simulink model "WBR_Simulator"  (R2023b)
settings: Solver=FixedStepAuto  StartTime=0.0  StopTime=60  FixedStep=0.001  MaxStep=0.001
undefined symbols (not defined in the file or in its folder): DiscIntNeverNeededParam, magnitude, robot_stats, SIMPARAM, X, Y, Z
libraries: sm_lib x73, nesl_utility x50, simulink x17, slpidlib x6, dsparch4 x2
(part 1 of 7)
settings Model: Creator=User  LastModifiedBy=User

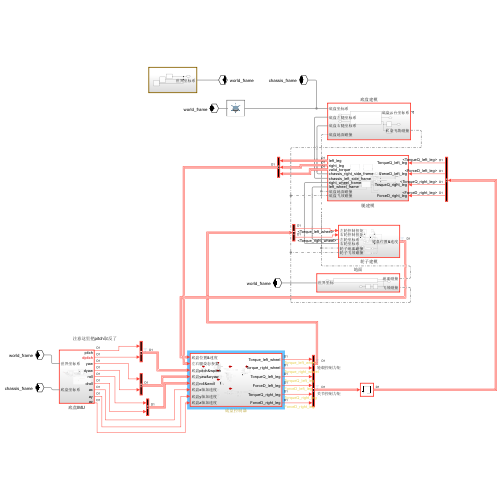
[thumbnail: Simulink's stored preview of the top-level diagram]
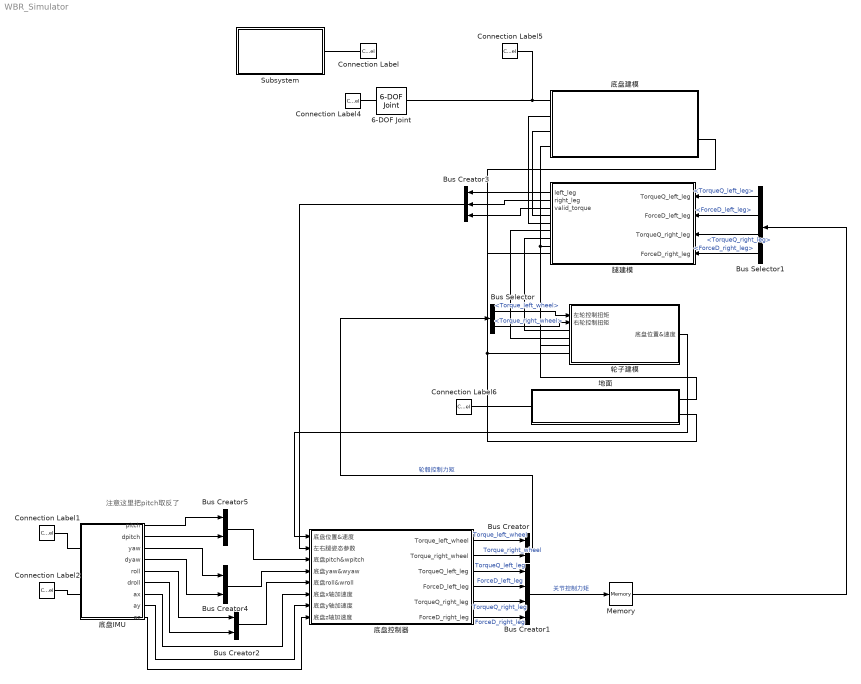
== system WBR_Simulator ==
  note: 注意这里把pitch取反了
  6-DOF Joint : sm_lib/Joints/6-DOF Joint  JointMode=Normal  SenseConstraintForce=off  SenseConstraintForceX=off  SenseConstraintForceY=off  SenseConstraintForceZ=off  SenseConstraintTorque=off  SenseConstraintTorqueX=off  SenseConstraintTorqueY=off  SenseConstraintTorqueZ=off  SenseTotalForce=off  SenseTotalForceX=off  SenseTotalForceY=off  SenseTotalForceZ=off  SenseTotalTorque=off  SenseTotalTorqueX=off  SenseTotalTorqueY=off  SenseTotalTorqueZ=off  CompositeWrenchDir=FollowerOnBase  CompositeWrenchFrame=BaseFrame  PxEquilibriumPosition=0  PxEquilibriumPositionUnits=m  PxSpringStiffness=0  PxSpringStiffnessUnits=N/m  PxDampingCoefficient=0  PxDampingCoefficientUnits=N/(m/s)  PxTorqueActuationMode=NoTorque  PxMotionActuationMode=ComputedMotion  PxSensePosition=off  PxSenseVelocity=off  PxSenseAcceleration=off  PxSenseTorqueForce=off  PxSenseLowerLimitTorqueForce=off  PxSenseUpperLimitTorqueForce=off  PxLowerLimitSpecify=off  PxLowerLimitBound=-1  PxLowerLimitBoundUnits=m  PxLowerLimitStiffness=1e6  PxLowerLimitStiffnessUnits=N/m  PxLowerLimitDamping=1e3  PxLowerLimitDampingUnits=N/(m/s)  PxLowerLimitTransitionRegionWidth=1e-4  PxLowerLimitTransitionRegionWidthUnits=m  PxUpperLimitSpecify=off  PxUpperLimitBound=1  PxUpperLimitBoundUnits=m  PxUpperLimitStiffness=1e6  PxUpperLimitStiffnessUnits=N/m  PxUpperLimitDamping=1e3  PxUpperLimitDampingUnits=N/(m/s)  PxUpperLimitTransitionRegionWidth=1e-4  PxUpperLimitTransitionRegionWidthUnits=m  PxPositionTargetSpecify=off  PxPositionTargetPriority=High  PxPositionTargetValue=0  PxPositionTargetValueUnits=m  PxVelocityTargetSpecify=on  PxVelocityTargetPriority=High  PxVelocityTargetValue=SIMPARAM.init_vx  PxVelocityTargetValueUnits=m/s  PyEquilibriumPosition=0  PyEquilibriumPositionUnits=m  PySpringStiffness=0  PySpringStiffnessUnits=N/m  PyDampingCoefficient=0  PyDampingCoefficientUnits=N/(m/s)  PyTorqueActuationMode=NoTorque  PyMotionActuationMode=ComputedMotion  PySensePosition=off  PySenseVelocity=off  PySenseAcceleration=off  PySenseTorqueForce=off  PySenseLowerLimitTorqueForce=off  PySenseUpperLimitTorqueForce=off  PyLowerLimitSpecify=off  PyLowerLimitBound=-1  PyLowerLimitBoundUnits=m  PyLowerLimitStiffness=1e6  PyLowerLimitStiffnessUnits=N/m  PyLowerLimitDamping=1e3  PyLowerLimitDampingUnits=N/(m/s)  PyLowerLimitTransitionRegionWidth=1e-4  PyLowerLimitTransitionRegionWidthUnits=m  PyUpperLimitSpecify=off  PyUpperLimitBound=1  PyUpperLimitBoundUnits=m  PyUpperLimitStiffness=1e6  PyUpperLimitStiffnessUnits=N/m  PyUpperLimitDamping=1e3  PyUpperLimitDampingUnits=N/(m/s)  PyUpperLimitTransitionRegionWidth=1e-4  PyUpperLimitTransitionRegionWidthUnits=m  PyPositionTargetSpecify=off  PyPositionTargetPriority=High  PyPositionTargetValue=0  PyPositionTargetValueUnits=m  PyVelocityTargetSpecify=off  PyVelocityTargetPriority=High  PyVelocityTargetValue=0  PyVelocityTargetValueUnits=m/s  PzEquilibriumPosition=0  PzEquilibriumPositionUnits=m  PzSpringStiffness=0  PzSpringStiffnessUnits=N/m  PzDampingCoefficient=0  PzDampingCoefficientUnits=N/(m/s)  PzTorqueActuationMode=NoTorque  PzMotionActuationMode=ComputedMotion  PzSensePosition=off  PzSenseVelocity=off  PzSenseAcceleration=off  PzSenseTorqueForce=off  PzSenseLowerLimitTorqueForce=off  PzSenseUpperLimitTorqueForce=off  PzLowerLimitSpecify=off  PzLowerLimitBound=-1  PzLowerLimitBoundUnits=m  PzLowerLimitStiffness=1e6  PzLowerLimitStiffnessUnits=N/m  PzLowerLimitDamping=1e3  PzLowerLimitDampingUnits=N/(m/s)  PzLowerLimitTransitionRegionWidth=1e-4  PzLowerLimitTransitionRegionWidthUnits=m  PzUpperLimitSpecify=off  PzUpperLimitBound=1  PzUpperLimitBoundUnits=m  PzUpperLimitStiffness=1e6  PzUpperLimitStiffnessUnits=N/m  PzUpperLimitDamping=1e3  PzUpperLimitDampingUnits=N/(m/s)  PzUpperLimitTransitionRegionWidth=1e-4  PzUpperLimitTransitionRegionWidthUnits=m  PzPositionTargetSpecify=on  PzPositionTargetPriority=High  PzPositionTargetValue=SIMPARAM.init_z  PzPositionTargetValueUnits=m  PzVelocityTargetSpecify=off  PzVelocityTargetPriority=High  PzVelocityTargetValue=0  PzVelocityTargetValueUnits=m/s  SphEqPosRotationMethod=None  SphEqPosRotationAngleUnits=deg  SphEqPosRotationStandardAxis=+Z  SphEqPosRotationAngle=0.0  SphEqPosRotationArbitraryAxis=[0 0 1]  SphEqPosFollAlignAxisA=+X  SphEqPosBaseAlignAxisA=+Y  SphEqPosFollAlignAxisB=+Y  SphEqPosBaseAlignAxisB=+Z  SphEqPosRotationSequenceAxes=FollowerAxes  SphEqPosRotationSequence=XYX  SphEqPosRotationSequenceAngles=[0 0 0]  SphEqPosRotationSequenceAnglesUnits=deg  SphEqPosRotationMatrix=[1 0 0; 0 1 0; 0 0 1]  SphEqPosQuaternion=[1 0 0 0]  SphSpringStiffness=0  SphSpringStiffnessUnits=N*m/deg  SphDampingCoefficient=0  SphDampingCoefficientUnits=N*m/(deg/s)  SphActuateTorqueX=off  SphActuateTorqueY=off  SphActuateTorqueZ=off  SphActuateTorque=off  SphTorqueActuationMode=NoTorque  SphMotionActuationMode=ComputedMotion  SphActuationFrame=FollowerFrame  SphSensePosition=off  SphSenseVelocityX=off  SphSenseVelocityY=off  SphSenseVelocityZ=off  SphSenseVelocity=off  SphSenseAccelerationX=off  SphSenseAccelerationY=off  SphSenseAccelerationZ=off  SphSenseAcceleration=off  SphSenseTorqueX=off  SphSenseTorqueY=off  SphSenseTorqueZ=off  SphSenseTorqueForce=off  SphSenseLowerLimitTorqueMag=off  SphSenseUpperLimitTorqueMag=off  SphSensingFrame=BaseFrame  SphLowerLimitSpecify=off  SphLowerLimitBound=15  SphLowerLimitBoundUnits=deg  SphLowerLimitStiffness=1e4  SphLowerLimitStiffnessUnits=N*m/deg  SphLowerLimitDamping=10  SphLowerLimitDampingUnits=N*m/(deg/s)  SphLowerLimitTransitionRegionWidth=0.1  SphLowerLimitTransitionRegionWidthUnits=deg  SphUpperLimitSpecify=off  SphUpperLimitBound=45  SphUpperLimitBoundUnits=deg  SphUpperLimitStiffness=1e4  SphUpperLimitStiffnessUnits=N*m/deg  SphUpperLimitDamping=10  SphUpperLimitDampingUnits=N*m/(deg/s)  SphUpperLimitTransitionRegionWidth=0.1  SphUpperLimitTransitionRegionWidthUnits=deg  SphPositionTargetRotationMethod=StandardAxis  SphPositionTargetRotationAngleUnits=rad  SphPositionTargetRotationStandardAxis=+Y  SphPositionTargetRotationAngle=0  SphPositionTargetRotationArbitraryAxis=[0 0 1]  SphPositionTargetFollAlignAxisA=+X  SphPositionTargetBaseAlignAxisA=+Y  SphPositionTargetFollAlignAxisB=+Y  SphPositionTargetBaseAlignAxisB=+Z  SphPositionTargetRotationSequenceAxes=FollowerAxes  SphPositionTargetRotationSequence=XYX  SphPositionTargetRotationSequenceAngles=[0 0 0]  SphPositionTargetRotationSequenceAnglesUnits=deg  SphPositionTargetRotationMatrix=[1 0 0; 0 1 0; 0 0 1]  SphPositionTargetQuaternion=[1 0 0 0]  SphPositionTargetSpecify=on  SphPositionTargetPriority=High  SphVelocityTargetValue=[0 0 0]  SphVelocityTargetValueUnits=deg/s  SphVelocityTargetSpecify=off  SphVelocityTargetPriority=High  SphVelocityTargetInFollowerFrame=on
  Bus Creator{,2,4..5} (4 alike) : BusCreator  Inputs=2
  Bus Creator1 : BusCreator  Inputs=4
  Bus Creator3 : BusCreator  Inputs=3
  Bus Selector : BusSelector  OutputSignals=Torque_left_wheel,Torque_right_wheel
  Bus Selector1 : BusSelector  OutputSignals=TorqueQ_left_leg,ForceD_left_leg,TorqueQ_right_leg,ForceD_right_leg
  Connection Label{,1,4,6} (4 alike) : ConnectionLabel  Label=world_frame
  Connection Label2 : ConnectionLabel  Label=chassis_frame
  Connection Label5 : ConnectionLabel  Label=chassis_frame
  Memory : Memory
  Subsystem : Subsystem
  地面 : Subsystem
  底盘IMU : Subsystem
  底盘建模 : Subsystem
  底盘控制器 : Subsystem
  腿建模 : Subsystem
  轮子建模 : Subsystem
  wires:
  轮子建模/1(底盘位置&速度) -> 底盘控制器/1(底盘位置&速度)
  腿建模/1(left_leg) -> Bus Creator3/1
  腿建模/2(right_leg) -> Bus Creator3/2
  腿建模/3(valid_torque) -> Bus Creator3/3
  Bus Creator3/1 -> 底盘控制器/2(左右腿姿态参数)
  底盘IMU/1(pitch) -> Bus Creator5/1
  底盘IMU/2(dpitch) -> Bus Creator5/2
  底盘IMU/3(yaw) -> Bus Creator4/1
  底盘IMU/4(dyaw) -> Bus Creator4/2
  Bus Creator4/1 -> 底盘控制器/4(底盘yaw&wyaw)
  Bus Creator5/1 -> 底盘控制器/3(底盘pitch&wpitch)
  底盘控制器/3(TorqueQ_left_leg) -> Bus Creator1/1  "TorqueQ_left_leg"
  底盘控制器/4(ForceD_left_leg) -> Bus Creator1/2  "ForceD_left_leg"
  底盘控制器/5(TorqueQ_right_leg) -> Bus Creator1/3  "TorqueQ_right_leg"
  底盘控制器/6(ForceD_right_leg) -> Bus Creator1/4  "ForceD_right_leg"
  底盘控制器/2(Torque_right_wheel) -> Bus Creator/2  "Torque_right_wheel"
  底盘控制器/1(Torque_left_wheel) -> Bus Creator/1  "Torque_left_wheel"
  Bus Selector1/1 -> 腿建模/1(TorqueQ_left_leg)  "<TorqueQ_left_leg>"
  Bus Selector1/2 -> 腿建模/2(ForceD_left_leg)  "<ForceD_left_leg>"
  Bus Selector1/3 -> 腿建模/3(TorqueQ_right_leg)  "<TorqueQ_right_leg>"
  Bus Selector1/4 -> 腿建模/4(ForceD_right_leg)  "<ForceD_right_leg>"
  Bus Creator/1 -> Bus Selector/1  "轮毂控制力矩"
  Bus Selector/1 -> 轮子建模/1(左轮控制扭矩)  "<Torque_left_wheel>"
  Bus Selector/2 -> 轮子建模/2(右轮控制扭矩)  "<Torque_right_wheel>"
  Bus Creator1/1 -> Memory/1  "关节控制力矩"
  底盘IMU/5(roll) -> Bus Creator2/1
  底盘IMU/6(droll) -> Bus Creator2/2
  Bus Creator2/1 -> 底盘控制器/5(底盘roll&wroll)
  底盘IMU/9(az) -> 底盘控制器/8(底盘z轴加速度)
  底盘IMU/7(ax) -> 底盘控制器/6(底盘x轴加速度)
  底盘IMU/8(ay) -> 底盘控制器/7(底盘y轴加速度)
  Memory/1 -> Bus Selector1/1
  connections:
  Connection Label/LConn1 -- Subsystem/RConn1
  Connection Label1/LConn1 -- 底盘IMU/LConn1
  底盘IMU/LConn2 -- Connection Label2/LConn1
  Connection Label4/LConn1 -- 6-DOF Joint/LConn1
  底盘建模/RConn1 -- Connection Label5/LConn1 -- 6-DOF Joint/RConn1
  腿建模/RConn5 -- 地面/LConn1 -- 轮子建模/LConn3 -- 底盘建模/RConn4
  腿建模/RConn2 -- 底盘建模/RConn2
  腿建模/RConn1 -- 底盘建模/RConn3
  腿建模/RConn4 -- 轮子建模/LConn1
  腿建模/RConn3 -- 轮子建模/LConn2
  地面/RConn1 -- Connection Label6/LConn1
  轮子建模/LConn4 -- 底盘建模/LConn2 -- 腿建模/RConn6 -- 地面/LConn2

== system WBR_Simulator/Subsystem ==
  Mechanism Configuration : sm_lib/Utilities/Mechanism Configuration  UniformGravity=Constant  GravityVector=[0 0 -9.8]  GravityVectorUnits=m/s^2  LinearizationDelta=0.001  JointModeTransitionNonlinearIterations=2
  Solver Configuration : nesl_utility/Solver Configuration  PhysicalDomain=network_engine_domain  SubClassName=solver  LeftPortType=input  RightPortType=generic  Tones=[]  Harmonics=[]  SimulateNoise=off  Profile=off  UseLocalSampling=off  EnableSwitchedLinearOptims=on  FrequencyDomain=off  UseCCode=off  RelTol=0.001  AbsTol=1e-06  MinStep=1e-09  ToWorkspace=off  RevertToSquareIcSolve=off  NumHomotopyIterations=100  PhasorMode=off  PhasorModeNumHarmonics=1  ConsistencySolver=NEWTON_FTOL  IndexReductionMethod=DerivativeReplacement  DoDC=off  ResidualTolerance=1e-06  ConsistencyTolSource=GLOBAL  ConsistencyAbsTol=0.001  ConsistencyRelTol=0.001  ConsistencyTolFactor=0.001  UseLocalSolver=off  LocalSolverChoice=NE_BACKWARD_EULER_ADVANCER  ResolveIndetEquations=on  FunctionEvalNumThread=1  LocalSolverSampleTime=0.001  DoFixedCost=off  MaxNonlinIter=3  MaxModeIter=2  ComputeImpulses=off  ImpulseIterations=2  LinearAlgebra=auto  LinearAlgebraNumThread=0  EquationFormulation=NE_TIME_EF  DelaysMemoryBudget=1024  AutomaticFiltering=on  FilteringTimeConstant=0.001  PartitionStorageMethod=AS_NEEDED  PartitionMemoryBudget=1024  PartitionMethod=ROBUST  MultibodyUseLocalSolver=off  MultibodyLocalSolverChoice=ODE1  MultibodyLocalSolverSampleTime=0.001
  World Frame : sm_lib/Frames and Transforms/World Frame
  世界坐标系 : PMIOPort  Side=Right
  connections:
  Solver Configuration/RConn1 -- Mechanism Configuration/RConn1 -- World Frame/RConn1 -- 世界坐标系/RConn1

== system WBR_Simulator/地面 ==
  Brick Solid : sm_lib/Body Elements/Brick Solid  GraphicAmbientColor=[0.15 0.15 0.15 1.0]  BasedOnType=Density  BrickDimensions=[3 100 0.1]  BrickDimensionsUnits=m  CenterOfMass=[0 0 0]  CenterOfMassUnits=m  GraphicDiffuseColor=[0.5 0.5 0.5]  Density=1000  DensityUnits=kg/m^3  DoExposeReferenceFrame=on  GraphicEmissiveColor=[0.0 0.0 0.0 1.0]  ExportEntireGeometry=on  SerializedFrames=<Frames/>  MarkerShape=Sphere  MarkerSize=10  GraphicType=FromGeometry  InertiaType=CalculateFromGeometry  Mass=1  MassUnits=kg  MomentsOfInertia=[1 1 1]  MomentsOfInertiaUnits=kg*m^2  GraphicOpacity=1.0  ProductsOfInertia=[0 0 0]  ProductsOfInertiaUnits=kg*m^2  GraphicShininess=75  GraphicSpecularColor=[0.5 0.5 0.5 1.0]  GraphicVisPropType=SimpleVisualProperties
  Rigid Transform : sm_lib/Frames and Transforms/Rigid Transform  TranslationMethod=Cartesian  TranslationStandardOffset=1.5  TranslationStandardOffsetUnits=m  TranslationStandardAxis=-X  TranslationCartesianOffset=[-1 0 0.25]  TranslationCartesianOffsetUnits=m  TranslationROffset=0  TranslationROffsetUnits=m  TranslationZOffset=0  TranslationZOffsetUnits=m  TranslationThetaOffset=0  TranslationThetaOffsetUnits=deg  RotationMethod=StandardAxis  RotationAngleUnits=deg  RotationStandardAxis=+Y  RotationAngle=17  RotationArbitraryAxis=[0 0 1]  FollAlignAxisA=+X  BaseAlignAxisA=+Y  FollAlignAxisB=+Y  BaseAlignAxisB=+Z  RotationSequenceAxes=FollowerAxes  RotationSequence=XYX  RotationSequenceAngles=[0 0 0]  RotationSequenceAnglesUnits=deg  RotationMatrix=[1 0 0; 0 1 0; 0 0 1]  Quaternion=[1 0 0 0]
  ground : sm_lib/Body Elements/Brick Solid  GraphicAmbientColor=[0.15 0.15 0.15 1.0]  BasedOnType=Density  BrickDimensions=[50 100 0.1]  BrickDimensionsUnits=m  CenterOfMass=[0 0 0]  CenterOfMassUnits=m  GraphicDiffuseColor=[0.0 0.4 0.4]  Density=114514  DensityUnits=kg/m^3  DoExposeReferenceFrame=on  GraphicEmissiveColor=[0.0 0.0 0.0 1.0]  ExportEntireGeometry=on  SerializedFrames=<Frames><Frame><Id>Frame1</Id><Value><Name>feipo</Name><Origin><Source>ReferenceFrame</Source><FeatureName></FeatureName></Origin><PrimaryAxis><DefinedDirection>+Z</DefinedDirection><Source>ReferenceFrame</Source><SourceDirection>+Z</SourceDirection><FeatureName></FeatureName></PrimaryAxis><SecondaryAxis><DefinedDirection>+X</DefinedDirection><Source>ReferenceFrame</Source><SourceDirection>+X</SourceDirection><FeatureName></FeatureName></SecondaryAxis></Value></Frame></Frames>  MarkerShape=Sphere  MarkerSize=10  GraphicType=FromGeometry  InertiaType=CalculateFromGeometry  Mass=0  MassUnits=kg  MomentsOfInertia=[1 1 1]  MomentsOfInertiaUnits=kg*m^2  GraphicOpacity=0.1  ProductsOfInertia=[0 0 0]  ProductsOfInertiaUnits=kg*m^2  GraphicShininess=0  GraphicSpecularColor=[1 1 1 1.0]  GraphicVisPropType=SimpleVisualProperties
  世界坐标 : PMIOPort  Side=Right
  地面碰撞 : PMIOPort  Port=2  Side=Left
  飞坡碰撞 : PMIOPort  Port=3  Side=Left
  connections:
  Rigid Transform/RConn1 -- ground/LConn1
  ground/RConn1 -- 世界坐标/RConn1
  Brick Solid/RConn1 -- Rigid Transform/LConn1
  Brick Solid/LConn1 -- 地面碰撞/RConn1
  ground/LConn2 -- 飞坡碰撞/RConn1

== system WBR_Simulator/底盘IMU ==
  note: 输出结果应遵循右手系
      | Z
      | |
      | |
      | |
      | | X: IN FRONT OF YOUR HEAD
      | | /
      | | /
      | Y <-------ROBOT
  Discrete Derivative : simulink/Discrete/Discrete Derivative  gainval=1.0  ICPrevScaledInput=0.0  OutMin=[]  OutMax=[]  OutDataType=fixdt(1, 16)  OutScaling=2^-10  DoSatur=off
  Discrete Derivative1 : simulink/Discrete/Discrete Derivative  gainval=1.0  ICPrevScaledInput=0.0  OutMin=[]  OutMax=[]  OutDataType=fixdt(1, 16)  OutScaling=2^-10  DoSatur=off
  Discrete Derivative2 : simulink/Discrete/Discrete Derivative  gainval=1.0  ICPrevScaledInput=0.0  OutMin=[]  OutMax=[]  OutDataType=fixdt(1, 16)  OutScaling=2^-10  DoSatur=off
  MATLAB Function1 : MATLAB Function  TreatAsAtomicUnit=on
  PS-Simulink Converter{1..3,12,14} (5 alike) : nesl_utility/PS-Simulink Converter  PhysicalDomain=network_engine_domain  SubClassName=ps_output  LeftPortType=input  RightPortType=output  PseudoPeriodic=off  Frequencies=[]  VectorFormat=1-D array  Unit=inherit  AffineConversion=off
  Transform Sensor1 : sm_lib/Frames and Transforms/Transform Sensor  MeasurementFrame=World  RotationSequence=XYX  SenseAngle=off  SenseAxis=off  SenseQ=on  SenseR=off  SenseRotationSequence=off  SenseOmegaX=off  SenseOmegaY=off  SenseOmegaZ=on  SenseOmega=off  SenseQDot=off  SenseRDot=off  SenseRotationSequenceDot=off  SenseAlphaX=off  SenseAlphaY=off  SenseAlphaZ=off  SenseAlpha=off  SenseQDDot=off  SenseRDDot=off  SenseX=off  SenseY=off  SenseZ=off  SenseXYZ=off  SenseRad=off  SenseAzim=off  SenseDist=off  SenseInc=off  SenseXDot=off  SenseYDot=off  SenseZDot=off  SenseXYZDot=off  SenseRadDot=off  SenseAzimDot=off  SenseDistDot=off  SenseIncDot=off  SenseXDDot=on  SenseYDDot=on  SenseZDDot=on  SenseXYZDDot=off  SenseRadDDot=off  SenseAzimDDot=off  SenseDistDDot=off  SenseIncDDot=off
  Zero-Order Hold{,1..4} (5 alike) : ZeroOrderHold  SampleTime=0.001
  世界坐标系 : PMIOPort  Side=Left
  底盘坐标系 : PMIOPort  Port=2  Side=Left
  pitch : Outport
  dpitch : Outport  Port=2
  yaw : Outport  Port=3
  dyaw : Outport  Port=4
  roll : Outport  Port=5
  droll : Outport  Port=6
  ax : Outport  Port=7
  ay : Outport  Port=8
  az : Outport  Port=9
  wires:
  MATLAB Function1/1(pitch) -> Discrete Derivative2/1, pitch/1  "pitch"
  MATLAB Function1/2(yaw) -> Discrete Derivative1/1, yaw/1
  PS-Simulink Converter12/1 -> Zero-Order Hold4/1
  Discrete Derivative2/1 -> dpitch/1  "dpitch"
  Discrete Derivative1/1 -> dyaw/1  "dyaw"
  PS-Simulink Converter1/1 -> Zero-Order Hold2/1
  MATLAB Function1/3(roll) -> Discrete Derivative/1, roll/1
  Discrete Derivative/1 -> droll/1  "droll"
  PS-Simulink Converter3/1 -> Zero-Order Hold1/1
  PS-Simulink Converter2/1 -> Zero-Order Hold/1
  Zero-Order Hold/1 -> ax/1
  Zero-Order Hold1/1 -> ay/1
  Zero-Order Hold2/1 -> az/1
  PS-Simulink Converter14/1 -> Zero-Order Hold3/1  "wyaw"
  Zero-Order Hold4/1 -> MATLAB Function1/1(quat_theta)
  connections:
  Transform Sensor1/RConn3 -- PS-Simulink Converter14/LConn1
  Transform Sensor1/RConn2 -- PS-Simulink Converter12/LConn1
  Transform Sensor1/LConn1 -- 世界坐标系/RConn1
  底盘坐标系/RConn1 -- Transform Sensor1/RConn1
  Transform Sensor1/RConn6 -- PS-Simulink Converter1/LConn1
  PS-Simulink Converter3/LConn1 -- Transform Sensor1/RConn5
  Transform Sensor1/RConn4 -- PS-Simulink Converter2/LConn1

== system WBR_Simulator/底盘建模 ==
  Spatial Contact Force1 : sm_lib/Forces and Torques/Spatial Contact Force  SenseContactBaseRotation=off  SenseContactBaseTranslation=off  CoefficientOfDynamicFriction=0.3  CoefficientOfStaticFriction=0.5  NormalDamping=1e6  NormalDampingUnits=N/(m/s)  SenseContactSignal=off  NormalStiffness=1e6  NormalStiffnessUnits=N/m  FrictionalCriticalVelocity=1e-3  FrictionalCriticalVelocityUnits=m/s  ZeroCrossDetectContactStartAndEnd=off  SenseContactFollowerRotation=off  SenseContactFollowerTranslation=off  FrictionType=SmoothStickSlip  SenseFrictionalForceMagnitude=off  SenseNormalForceMagnitude=off  NormalForceType=SmoothSpringDamper  SenseNormalVelocity=off  SensePenetrationDepth=off  SenseSeparationDistance=off  SenseTangentialVelocity=off  NormalTransitionRegionWidth=1e-4  NormalTransitionRegionWidthUnits=m
  Spatial Contact Force2 : sm_lib/Forces and Torques/Spatial Contact Force  SenseContactBaseRotation=off  SenseContactBaseTranslation=off  CoefficientOfDynamicFriction=0.3  CoefficientOfStaticFriction=0.5  NormalDamping=1e6  NormalDampingUnits=N/(m/s)  SenseContactSignal=off  NormalStiffness=1e6  NormalStiffnessUnits=N/m  FrictionalCriticalVelocity=1e-3  FrictionalCriticalVelocityUnits=m/s  ZeroCrossDetectContactStartAndEnd=off  SenseContactFollowerRotation=off  SenseContactFollowerTranslation=off  FrictionType=SmoothStickSlip  SenseFrictionalForceMagnitude=off  SenseNormalForceMagnitude=off  NormalForceType=SmoothSpringDamper  SenseNormalVelocity=off  SensePenetrationDepth=off  SenseSeparationDistance=off  SenseTangentialVelocity=off  NormalTransitionRegionWidth=1e-4  NormalTransitionRegionWidthUnits=m
  底盘 : sm_lib/Body Elements/Brick Solid  GraphicAmbientColor=[0.15 0.15 0.15 1.0]  BasedOnType=Mass  BrickDimensions=[robot_stats.chassis_length robot_stats.chassis_width robot_stats.chassis_height]  BrickDimensionsUnits=m  CenterOfMass=[0 0 0]  CenterOfMassUnits=m  GraphicDiffuseColor=[1.0 1.0 1.0]  Density=1000  DensityUnits=kg/m^3  DoExposeReferenceFrame=on  GraphicEmissiveColor=[0.0 0.0 0.0 1.0]  ExportEntireGeometry=on  SerializedFrames=<Frames><Frame><Id>Frame1</Id><Value><Name>right_hang</Name><Origin><Source>GeometricFeature</Source><FeatureName>-y -z curve</FeatureName></Origin><PrimaryAxis><DefinedDirection>-Z</DefinedDirection><Source>ReferenceFrame</Source><SourceDirection>+Z</SourceDirection><FeatureName></FeatureName></PrimaryAxis><SecondaryAxis><DefinedDirection>+X</DefinedDirection><Source>ReferenceFrame</Source><SourceDirection>+X</SourceDirection><FeatureName></FeatureName></SecondaryAxis></Value></Frame><Frame><Id>Frame2</Id><Value><Name>gimbal_base</Name><Origin><Source>GeometricFeature</Source><FeatureName>+z surface</FeatureName></Origin><PrimaryAxis><DefinedDirection>+Z</DefinedDirection><Source>ReferenceFrame</Source><SourceDirection>+Z</SourceDirection><FeatureName></FeatureName></PrimaryAxis><SecondaryAxis><DefinedDirection>+X</DefinedDirection><Source>ReferenceFrame</Source><SourceDirection>+X</SourceDirection><FeatureName></FeatureName></SecondaryAxis></Value></Frame><Frame><Id>Frame3</Id><Value><Name>left_hang</Name><Origin><Source>GeometricFeature</Source><FeatureName>+y -z curve</FeatureName></Origin><PrimaryAxis><DefinedDirection>-Z</DefinedDirection><Source>ReferenceFrame</Source><SourceDirection>+Z</SourceDirection><FeatureName></FeatureName></PrimaryAxis><SecondaryAxis><DefinedDirection>+X</DefinedDirection><Source>ReferenceFrame</Source><SourceDirection>+X</SourceDirection><FeatureName></FeatureName></SecondaryAxis></Value></Frame></Frames>  MarkerShape=Sphere  MarkerSize=10  GraphicType=FromGeometry  InertiaType=CalculateFromGeometry  Mass=robot_stats.mass_body  MassUnits=kg  MomentsOfInertia=[1 1 1]  MomentsOfInertiaUnits=kg*m^2  GraphicOpacity=1.0  ProductsOfInertia=[0 0 0]  ProductsOfInertiaUnits=kg*m^2  GraphicShininess=75  GraphicSpecularColor=[0.5 0.5 0.5 1.0]  GraphicVisPropType=SimpleVisualProperties
  底盘云台坐标系 : PMIOPort  Side=Left
  底盘飞坡碰撞 : PMIOPort  Port=2  Side=Left
  底盘坐标系 : PMIOPort  Port=3  Side=Right
  底盘左腿坐标系 : PMIOPort  Port=4  Side=Right
  底盘右腿坐标系 : PMIOPort  Port=5  Side=Right
  底盘地面碰撞 : PMIOPort  Port=6  Side=Right
  connections:
  底盘左腿坐标系/RConn1 -- 底盘/RConn2
  底盘/LConn2 -- 底盘云台坐标系/RConn1
  底盘坐标系/RConn1 -- 底盘/RConn1
  Spatial Contact Force2/RConn1 -- 底盘/LConn3 -- Spatial Contact Force1/RConn1
  底盘右腿坐标系/RConn1 -- 底盘/LConn1
  Spatial Contact Force2/LConn1 -- 底盘地面碰撞/RConn1
  底盘飞坡碰撞/RConn1 -- Spatial Contact Force1/LConn1
